simulink model "fir_arty_ip"  (R2026a)
settings: Solver=FixedStepDiscrete  StopTime=300  FixedStep=1
model workspace (MAT data in the model file):
  b = [0.125 0.375 0.375 0.125]
  f_noise = 0.4
  f_sig = 0.01
libraries: hdlsllib x2, simulink x1
settings Model: Creator=KoayXianCong  LastModifiedBy=KoayXianCong

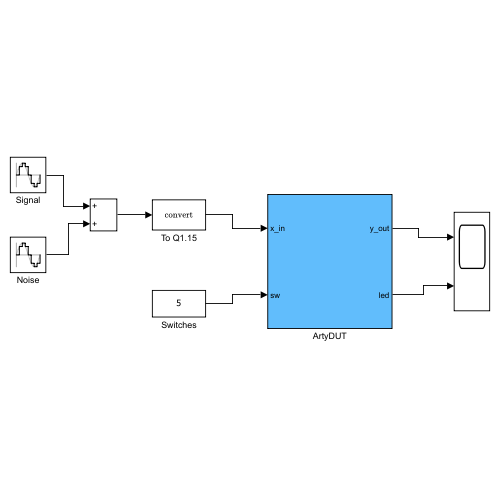
[thumbnail: Simulink's stored preview of the top-level diagram]
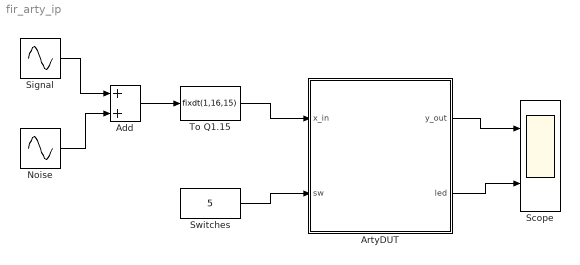
== system fir_arty_ip ==
  Add : Sum
  ArtyDUT : Subsystem
  Noise : Sin  Amplitude=0.4  Frequency=2*pi*f_noise  SampleTime=1
  Scope : Scope  NumInputPorts=2
  Signal : Sin  Amplitude=0.5  Frequency=2*pi*f_sig  SampleTime=1
  Switches : Constant  Value=5  OutDataTypeStr=fixdt(0,4,0)
  To Q1.15 : DataTypeConversion  OutDataTypeStr=fixdt(1,16,15)  RndMeth=Nearest
  wires:
  Signal/1 -> Add/1
  Noise/1 -> Add/2
  Add/1 -> To Q1.15/1
  To Q1.15/1 -> ArtyDUT/1(x_in)
  Switches/1 -> ArtyDUT/2(sw)
  ArtyDUT/1(y_out) -> Scope/1
  ArtyDUT/2(led) -> Scope/2

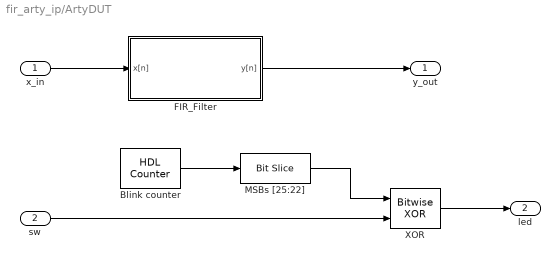
== system fir_arty_ip/ArtyDUT ==
  x_in : Inport
  sw : Inport  Port=2
  Blink counter : hdlsllib/Sources/HDL Counter  CountType=Count limited  CountInit=0  CountStep=1  CountMax=25  CountFromType=Initial value  CountFrom=0  CountResetPort=off  CountLoadPort=off  CountEnbPort=off  CountDirPort=off  CountHitOutputPort=off  CountDataType=Unsigned  CountWordLen=26  CountFracLen=0  CountSampTime=1
  FIR_Filter : Subsystem
  MSBs [25:22] : hdlsllib/Logic and Bit Operations/Bit Slice  lidx=25  ridx=22
  XOR : simulink/Logic and Bit Operations/Bitwise Operator  logicop=XOR  UseBitMask=off  NumInputPorts=2  BitMask=bin2dec('11011001')  BitMaskRealWorld=Stored Integer
  y_out : Outport
  led : Outport  Port=2
  wires:
  x_in/1 -> FIR_Filter/1(x[n])
  FIR_Filter/1(y[n]) -> y_out/1
  Blink counter/1 -> MSBs [25:22]/1
  MSBs [25:22]/1 -> XOR/1
  sw/1 -> XOR/2
  XOR/1 -> led/1

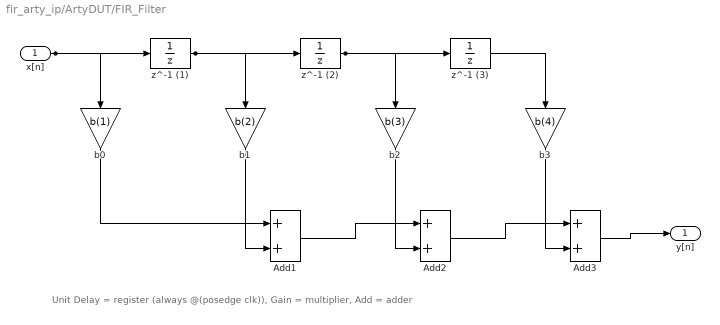
== system fir_arty_ip/ArtyDUT/FIR_Filter ==
  note: Unit Delay = register (always @(posedge clk)), Gain = multiplier, Add = adder
  x[n] : Inport
  Add1 : Sum  OutDataTypeStr=fixdt(1,19,18)
  Add2 : Sum  OutDataTypeStr=fixdt(1,19,18)
  Add3 : Sum  OutDataTypeStr=fixdt(1,19,18)
  b0 : Gain  Gain=b(1)  ParamDataTypeStr=fixdt(1,16,15)  OutDataTypeStr=fixdt(1,19,18)
  b1 : Gain  Gain=b(2)  ParamDataTypeStr=fixdt(1,16,15)  OutDataTypeStr=fixdt(1,19,18)
  b2 : Gain  Gain=b(3)  ParamDataTypeStr=fixdt(1,16,15)  OutDataTypeStr=fixdt(1,19,18)
  b3 : Gain  Gain=b(4)  ParamDataTypeStr=fixdt(1,16,15)  OutDataTypeStr=fixdt(1,19,18)
  z^-1 (1) : UnitDelay  SampleTime=-1
  z^-1 (2) : UnitDelay  SampleTime=-1
  z^-1 (3) : UnitDelay  SampleTime=-1
  y[n] : Outport
  wires:
  Add3/1 -> y[n]/1
  b3/1 -> Add3/2
  Add2/1 -> Add3/1
  b2/1 -> Add2/2
  Add1/1 -> Add2/1
  b1/1 -> Add1/2
  b0/1 -> Add1/1
  z^-1 (3)/1 -> b3/1
  z^-1 (2)/1 -> b2/1, z^-1 (3)/1
  z^-1 (1)/1 -> b1/1, z^-1 (2)/1
  x[n]/1 -> b0/1, z^-1 (1)/1
